simulink model "Shaddad_MCU"  (R2026b)
undefined symbols (not defined in the file): P, Ts
libraries: simulink x25
settings Model: Creator=aomar  LastModifiedBy=aomar

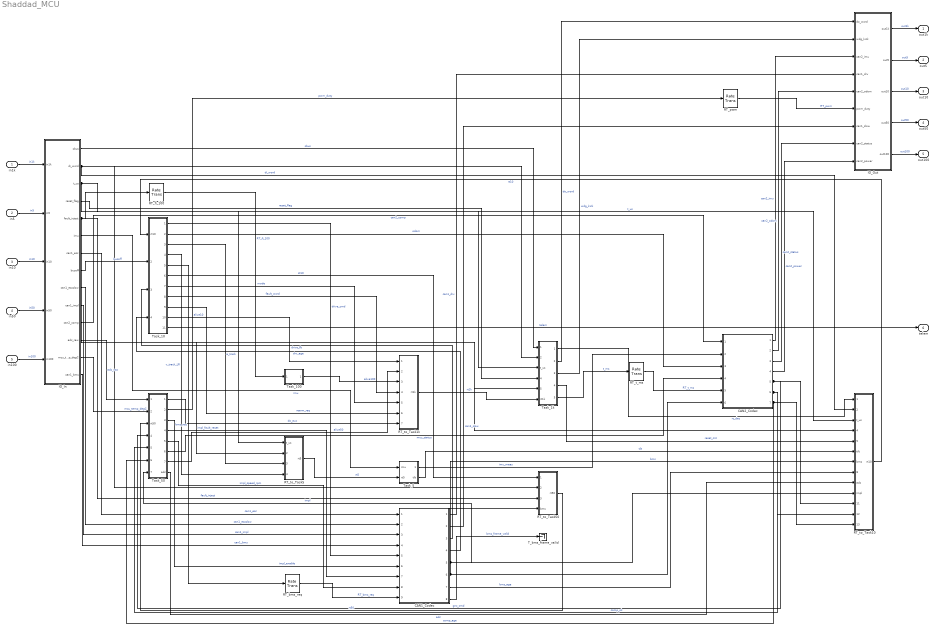
== system Shaddad_MCU ==
  in1k : Inport  OutDataTypeStr=Bus: Bus_McuIn1k  SampleTime=Ts.base  BusOutputAsStruct=on
  in5 : Inport  Port=2  OutDataTypeStr=Bus: Bus_McuIn5  SampleTime=Ts.imu  BusOutputAsStruct=on
  in10 : Inport  Port=3  OutDataTypeStr=Bus: Bus_McuIn10  SampleTime=Ts.ctrl  BusOutputAsStruct=on
  in50 : Inport  Port=4  OutDataTypeStr=Bus: Bus_McuIn50  SampleTime=Ts.comm  BusOutputAsStruct=on
  in100 : Inport  Port=5  OutDataTypeStr=Bus: Bus_McuIn100  SampleTime=Ts.hk  BusOutputAsStruct=on
  CAN1_Codec : Subsystem  ReferencedSubsystem=fw_can1_codec
  CAN2_Codec : Subsystem  ReferencedSubsystem=fw_can2_codec
  IO_In : Subsystem  Variant=on
  IO_Out : Subsystem  Variant=on
  RT_bms_req : RateTransition  OutPortSampleTime=Ts.comm
  RT_fi_100 : RateTransition  OutPortSampleTime=Ts.hk
  RT_pwm : RateTransition  OutPortSampleTime=Ts.ctrl
  RT_t_ms : RateTransition  OutPortSampleTime=Ts.comm
  RT_to_Task10 : Subsystem
  RT_to_Task1k : Subsystem
  RT_to_Task5 : Subsystem
  RT_to_Task50 : Subsystem
  T_bms_frame_valid : Terminator
  Task_10 : Subsystem  TreatAsAtomicUnit=on  SystemSampleTime=Ts.ctrl
  Task_100 : Subsystem  TreatAsAtomicUnit=on  SystemSampleTime=Ts.hk
  Task_1k : Subsystem  TreatAsAtomicUnit=on  SystemSampleTime=Ts.base
  Task_5 : Subsystem  TreatAsAtomicUnit=on  SystemSampleTime=Ts.imu
  Task_50 : Subsystem  TreatAsAtomicUnit=on  SystemSampleTime=Ts.comm
  out1k : Outport  OutDataTypeStr=Bus: Bus_McuOut1k  SampleTime=Ts.base  BusOutputAsStruct=on
  out5 : Outport  Port=2  OutDataTypeStr=Bus: Bus_McuOut5  SampleTime=Ts.imu  BusOutputAsStruct=on
  out10 : Outport  Port=3  OutDataTypeStr=Bus: Bus_McuOut10  SampleTime=Ts.ctrl  BusOutputAsStruct=on
  out50 : Outport  Port=4  OutDataTypeStr=Bus: Bus_McuOut50  SampleTime=Ts.comm  BusOutputAsStruct=on
  out100 : Outport  Port=5  OutDataTypeStr=Bus: Bus_McuOut100  SampleTime=Ts.hk  BusOutputAsStruct=on
  telem : Outport  Port=6  OutDataTypeStr=Bus: Bus_FwTelemetry  SampleTime=Ts.ctrl  BusOutputAsStruct=on
  wires:
  in1k/1 -> IO_In/1(in1k)  "in1k"
  in5/1 -> IO_In/2(in5)  "in5"
  in10/1 -> IO_In/3(in10)  "in10"
  in50/1 -> IO_In/4(in50)  "in50"
  in100/1 -> IO_In/5(in100)  "in100"
  IO_In/1(sbus) -> Task_1k/1(sbus)  "sbus"
  IO_In/2(di_word) -> RT_to_Task50/2(di_word), RT_to_Task10/2(di_word), Task_1k/2(di_word)  "di_word"
  IO_In/3(t_us) -> RT_to_Task5/1(t_us), RT_to_Task10/3(t_us), Task_1k/3(t_us)  "t_us"
  IO_In/4(reset_flag) -> Task_1k/4(reset_flag)  "reset_flag"
  IO_In/6(imu) -> Task_5/1(imu)  "imu"
  IO_In/7(can1_esc) -> CAN1_Codec/1  "can1_esc"
  IO_In/8(busoff) -> Task_10/2(busoff)  "busoff"
  IO_In/9(can1_escslow) -> CAN1_Codec/2  "can1_escslow"
  IO_In/10(can1_impl) -> CAN1_Codec/3  "can1_impl"
  IO_In/11(can2_comp) -> CAN2_Codec/1  "can2_comp"
  IO_In/13(mcu_temp_degC) -> Task_50/2(mcu_temp_degC)  "mcu_temp_degC"
  IO_In/14(can1_bms) -> CAN1_Codec/4  "can1_bms"
  RT_fi_100/1 -> Task_100/1(fault_inject)  "RT_fi_100"
  Task_10/1(drive_cmd) -> CAN1_Codec/5  "drive_cmd"
  Task_10/2(odom) -> CAN2_Codec/3  "odom"
  Task_10/3(a_track) -> RT_to_Task5/3(a_track)  "a_track"
  Task_10/4(v_track_LR) -> RT_to_Task5/4(v_track_LR)  "v_track_LR"
  Task_10/5(bms_req) -> RT_bms_req/1  "bms_req"
  Task_10/6(st10) -> RT_to_Task50/1(st10)  "st10"
  Task_10/7(mode) -> RT_to_Task1k/5(mode)  "mode"
  Task_10/8(fault_word) -> RT_to_Task1k/4(fault_word)  "fault_word"
  Task_10/9(rearm_req) -> RT_to_Task1k/6(rearm_req)  "rearm_req"
  Task_10/10(alive10) -> RT_to_Task1k/1(alive10)  "alive10"
  Task_10/11(telem) -> telem/1  "telem"
  Task_50/1(do_aux) -> RT_to_Task1k/7(do_aux)  "do_aux"
  Task_50/2(pwm_duty) -> RT_pwm/1  "pwm_duty"
  Task_50/3(impl_enable) -> CAN1_Codec/6  "impl_enable"
  Task_50/4(impl_fault_reset) -> CAN1_Codec/7  "impl_fault_reset"
  Task_50/5(impl_speed_rpm) -> CAN1_Codec/8  "impl_speed_rpm"
  Task_50/6(status) -> CAN2_Codec/4  "mcu_status"
  Task_50/7(alive50) -> RT_to_Task1k/2(alive50)  "alive50"
  Task_50/8(adc) -> RT_to_Task10/9(adc)  "adc"
  RT_bms_req/1 -> CAN1_Codec/9  "RT_bms_req"
  Task_100/1(alive100) -> RT_to_Task1k/3(alive100)  "alive100"
  RT_to_Task5/1(rt5) -> Task_5/2(rt5)  "rt5"
  RT_to_Task1k/1(rt1k) -> Task_1k/6(rt1k)  "rt1k"
  Task_5/1(imu_meas) -> CAN2_Codec/2  "imu_meas"
  Task_5/2(tilt) -> RT_to_Task10/6(tilt)  "tilt"
  CAN1_Codec/1 -> IO_Out/4(can1_drv)  "can1_drv"
  CAN1_Codec/2 -> IO_Out/7(can1_slow)  "can1_slow"
  CAN1_Codec/3 -> Task_10/3(drive_fb)  "drive_fb"
  CAN1_Codec/4 -> Task_10/4(drv_age)  "drv_age"
  CAN1_Codec/5 -> Task_50/7(impl), RT_to_Task10/10(impl)  "impl"
  CAN1_Codec/6 -> CAN2_Codec/6, RT_to_Task10/7(bms), RT_to_Task50/4(bms)  "bms"
  CAN1_Codec/7 -> RT_to_Task10/8(bms_age)  "bms_age"
  CAN1_Codec/8 -> T_bms_frame_valid/1  "bms_frame_valid"
  Task_1k/1(rc_dec) -> RT_to_Task10/1(rc_dec)  "rc_dec"
  Task_1k/2(do_word) -> IO_Out/1(do_word)  "do_word"
  Task_1k/3(wdg_kick) -> IO_Out/2(wdg_kick)  "wdg_kick"
  Task_1k/4(reset_cnt) -> RT_to_Task10/5(reset_cnt)  "reset_cnt"
  Task_1k/5(t_ms) -> RT_t_ms/1  "t_ms"
  RT_to_Task50/1(rt50) -> Task_50/3(rt50)  "rt50"
  RT_t_ms/1 -> CAN2_Codec/5  "RT_t_ms"
  RT_pwm/1 -> IO_Out/6(pwm_duty)  "RT_pwm"
  CAN2_Codec/1 -> IO_Out/3(can2_imu)  "can2_imu"
  CAN2_Codec/2 -> IO_Out/5(can2_odom)  "can2_odom"
  CAN2_Codec/3 -> IO_Out/8(can2_status)  "can2_status"
  CAN2_Codec/4 -> IO_Out/9(can2_power)  "can2_power"
  RT_to_Task10/1(rt10) -> Task_10/1(rt10)  "rt10"
  IO_Out/1(out1k) -> out1k/1  "out1k"
  IO_Out/2(out5) -> out5/1  "out5"
  IO_Out/3(out10) -> out10/1  "out10"
  IO_Out/4(out50) -> out50/1  "out50"
  IO_Out/5(out100) -> out100/1  "out100"
  CAN2_Codec/5 -> RT_to_Task10/11(gnc_cmd), Task_50/4(gnc_cmd)  "gnc_cmd"
  IO_In/5(fault_inject) -> RT_to_Task50/3(fault_inject), RT_to_Task5/2(fault_inject), RT_to_Task10/4(fault_inject), Task_1k/5(fault_inject), RT_fi_100/1  "fault_inject"
  IO_In/12(adc_raw) -> Task_50/1(adc_raw)  "adc_raw"
  CAN2_Codec/6 -> RT_to_Task10/12(comp_ok), Task_50/5(comp_ok)  "comp_ok"
  CAN2_Codec/7 -> RT_to_Task10/13(comp_age), Task_50/6(comp_age)  "comp_age"

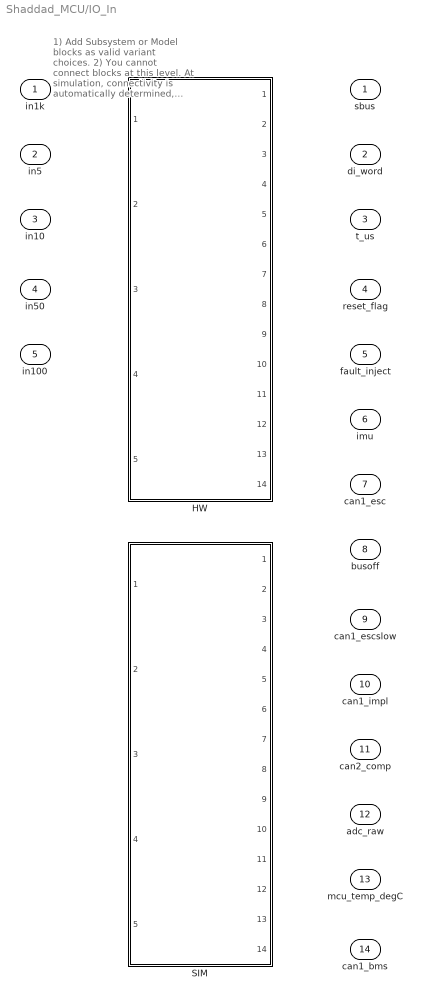
== system Shaddad_MCU/IO_In ==
  note: 1) Add Subsystem or Model blocks as valid variant choices.
      | 2) You cannot connect blocks at this level. At simulation, connectivity is automatically
      | determined, based on the active variant and port name matching.
  in1k : Inport
  in5 : Inport  Port=2
  in10 : Inport  Port=3
  in50 : Inport  Port=4
  in100 : Inport  Port=5
  HW : Subsystem  VariantControl=VC_TARGET == 1  ReferencedSubsystem=fw_io_in_hw
  SIM : Subsystem  VariantControl=VC_TARGET == 0  ReferencedSubsystem=fw_io_in_sim
  sbus : Outport
  di_word : Outport  Port=2
  t_us : Outport  Port=3
  reset_flag : Outport  Port=4
  fault_inject : Outport  Port=5
  imu : Outport  Port=6
  can1_esc : Outport  Port=7
  busoff : Outport  Port=8
  can1_escslow : Outport  Port=9
  can1_impl : Outport  Port=10
  can2_comp : Outport  Port=11
  adc_raw : Outport  Port=12
  mcu_temp_degC : Outport  Port=13
  can1_bms : Outport  Port=14

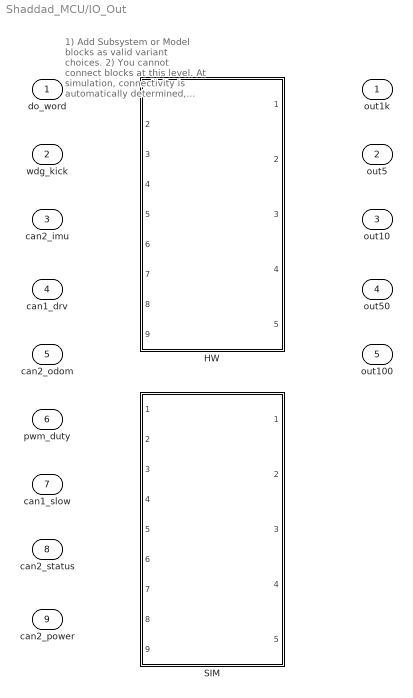
== system Shaddad_MCU/IO_Out ==
  note: 1) Add Subsystem or Model blocks as valid variant choices.
      | 2) You cannot connect blocks at this level. At simulation, connectivity is automatically
      | determined, based on the active variant and port name matching.
  do_word : Inport
  wdg_kick : Inport  Port=2
  can2_imu : Inport  Port=3
  can1_drv : Inport  Port=4
  can2_odom : Inport  Port=5
  pwm_duty : Inport  Port=6
  can1_slow : Inport  Port=7
  can2_status : Inport  Port=8
  can2_power : Inport  Port=9
  HW : Subsystem  VariantControl=VC_TARGET == 1  ReferencedSubsystem=fw_io_out_hw
  SIM : Subsystem  VariantControl=VC_TARGET == 0  ReferencedSubsystem=fw_io_out_sim
  out1k : Outport
  out5 : Outport  Port=2
  out10 : Outport  Port=3
  out50 : Outport  Port=4
  out100 : Outport  Port=5

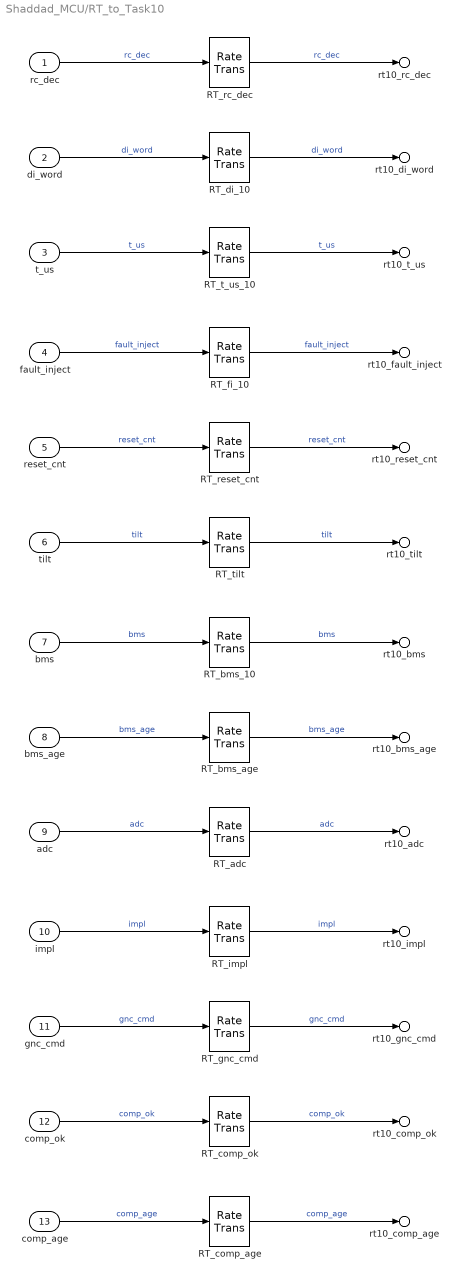
== system Shaddad_MCU/RT_to_Task10 ==
  rc_dec : Inport
  di_word : Inport  Port=2  OutDataTypeStr=uint16
  t_us : Inport  Port=3  OutDataTypeStr=uint32
  fault_inject : Inport  Port=4  OutDataTypeStr=uint32
  reset_cnt : Inport  Port=5  OutDataTypeStr=uint8
  tilt : Inport  Port=6
  bms : Inport  Port=7  OutDataTypeStr=Bus: Bus_BmsStatus
  bms_age : Inport  Port=8  OutDataTypeStr=single
  adc : Inport  Port=9
  impl : Inport  Port=10
  gnc_cmd : Inport  Port=11  OutDataTypeStr=Bus: Bus_GncCmd
  comp_ok : Inport  Port=12  OutDataTypeStr=boolean
  comp_age : Inport  Port=13  OutDataTypeStr=single
  RT_adc : RateTransition  OutPortSampleTime=Ts.ctrl
  RT_bms_10 : RateTransition  InitialCondition=P.ic.Bus_BmsStatus  OutPortSampleTime=Ts.ctrl
  RT_bms_age : RateTransition  OutPortSampleTime=Ts.ctrl
  RT_comp_age : RateTransition  OutPortSampleTime=Ts.ctrl
  RT_comp_ok : RateTransition  OutPortSampleTime=Ts.ctrl
  RT_di_10 : RateTransition  OutPortSampleTime=Ts.ctrl
  RT_fi_10 : RateTransition  OutPortSampleTime=Ts.ctrl
  RT_gnc_cmd : RateTransition  InitialCondition=P.ic.Bus_GncCmd  OutPortSampleTime=Ts.ctrl
  RT_impl : RateTransition  OutPortSampleTime=Ts.ctrl
  RT_rc_dec : RateTransition  OutPortSampleTime=Ts.ctrl
  RT_reset_cnt : RateTransition  OutPortSampleTime=Ts.ctrl
  RT_t_us_10 : RateTransition  OutPortSampleTime=Ts.ctrl
  RT_tilt : RateTransition  OutPortSampleTime=Ts.ctrl
  rt10_rc_dec : Outport  PortName=rt10  Element=rc_dec
  rt10_di_word : Outport  PortName=rt10  Element=di_word
  rt10_t_us : Outport  PortName=rt10  Element=t_us
  rt10_fault_inject : Outport  PortName=rt10  Element=fault_inject
  rt10_reset_cnt : Outport  PortName=rt10  Element=reset_cnt
  rt10_tilt : Outport  PortName=rt10  Element=tilt
  rt10_bms : Outport  PortName=rt10  Element=bms
  rt10_bms_age : Outport  PortName=rt10  Element=bms_age
  rt10_adc : Outport  PortName=rt10  Element=adc
  rt10_impl : Outport  PortName=rt10  Element=impl
  rt10_gnc_cmd : Outport  PortName=rt10  Element=gnc_cmd
  rt10_comp_ok : Outport  PortName=rt10  Element=comp_ok
  rt10_comp_age : Outport  PortName=rt10  Element=comp_age
  wires:
  rc_dec/1 -> RT_rc_dec/1  "rc_dec"
  di_word/1 -> RT_di_10/1  "di_word"
  t_us/1 -> RT_t_us_10/1  "t_us"
  fault_inject/1 -> RT_fi_10/1  "fault_inject"
  reset_cnt/1 -> RT_reset_cnt/1  "reset_cnt"
  tilt/1 -> RT_tilt/1  "tilt"
  bms/1 -> RT_bms_10/1  "bms"
  bms_age/1 -> RT_bms_age/1  "bms_age"
  adc/1 -> RT_adc/1  "adc"
  impl/1 -> RT_impl/1  "impl"
  gnc_cmd/1 -> RT_gnc_cmd/1  "gnc_cmd"
  comp_ok/1 -> RT_comp_ok/1  "comp_ok"
  comp_age/1 -> RT_comp_age/1  "comp_age"
  RT_rc_dec/1 -> rt10_rc_dec/1  "rc_dec"
  RT_di_10/1 -> rt10_di_word/1  "di_word"
  RT_t_us_10/1 -> rt10_t_us/1  "t_us"
  RT_fi_10/1 -> rt10_fault_inject/1  "fault_inject"
  RT_reset_cnt/1 -> rt10_reset_cnt/1  "reset_cnt"
  RT_tilt/1 -> rt10_tilt/1  "tilt"
  RT_bms_10/1 -> rt10_bms/1  "bms"
  RT_bms_age/1 -> rt10_bms_age/1  "bms_age"
  RT_adc/1 -> rt10_adc/1  "adc"
  RT_impl/1 -> rt10_impl/1  "impl"
  RT_gnc_cmd/1 -> rt10_gnc_cmd/1  "gnc_cmd"
  RT_comp_ok/1 -> rt10_comp_ok/1  "comp_ok"
  RT_comp_age/1 -> rt10_comp_age/1  "comp_age"

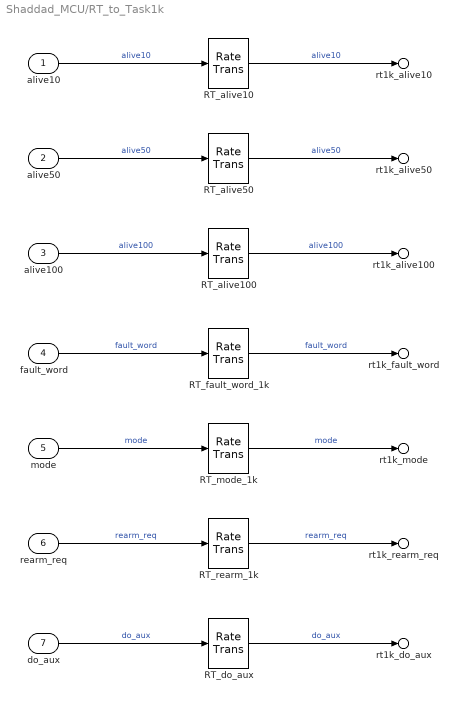
== system Shaddad_MCU/RT_to_Task1k ==
  alive10 : Inport  OutDataTypeStr=uint8
  alive50 : Inport  Port=2  OutDataTypeStr=uint8
  alive100 : Inport  Port=3  OutDataTypeStr=uint8
  fault_word : Inport  Port=4  OutDataTypeStr=uint32
  mode : Inport  Port=5  OutDataTypeStr=uint8
  rearm_req : Inport  Port=6  OutDataTypeStr=boolean
  do_aux : Inport  Port=7  OutDataTypeStr=uint32
  RT_alive10 : RateTransition  OutPortSampleTime=Ts.base
  RT_alive100 : RateTransition  OutPortSampleTime=Ts.base
  RT_alive50 : RateTransition  OutPortSampleTime=Ts.base
  RT_do_aux : RateTransition  OutPortSampleTime=Ts.base
  RT_fault_word_1k : RateTransition  OutPortSampleTime=Ts.base
  RT_mode_1k : RateTransition  OutPortSampleTime=Ts.base
  RT_rearm_1k : RateTransition  OutPortSampleTime=Ts.base
  rt1k_alive10 : Outport  PortName=rt1k  Element=alive10
  rt1k_alive50 : Outport  PortName=rt1k  Element=alive50
  rt1k_alive100 : Outport  PortName=rt1k  Element=alive100
  rt1k_fault_word : Outport  PortName=rt1k  Element=fault_word
  rt1k_mode : Outport  PortName=rt1k  Element=mode
  rt1k_rearm_req : Outport  PortName=rt1k  Element=rearm_req
  rt1k_do_aux : Outport  PortName=rt1k  Element=do_aux
  wires:
  alive10/1 -> RT_alive10/1  "alive10"
  alive50/1 -> RT_alive50/1  "alive50"
  alive100/1 -> RT_alive100/1  "alive100"
  fault_word/1 -> RT_fault_word_1k/1  "fault_word"
  mode/1 -> RT_mode_1k/1  "mode"
  rearm_req/1 -> RT_rearm_1k/1  "rearm_req"
  do_aux/1 -> RT_do_aux/1  "do_aux"
  RT_alive10/1 -> rt1k_alive10/1  "alive10"
  RT_alive50/1 -> rt1k_alive50/1  "alive50"
  RT_alive100/1 -> rt1k_alive100/1  "alive100"
  RT_fault_word_1k/1 -> rt1k_fault_word/1  "fault_word"
  RT_mode_1k/1 -> rt1k_mode/1  "mode"
  RT_rearm_1k/1 -> rt1k_rearm_req/1  "rearm_req"
  RT_do_aux/1 -> rt1k_do_aux/1  "do_aux"

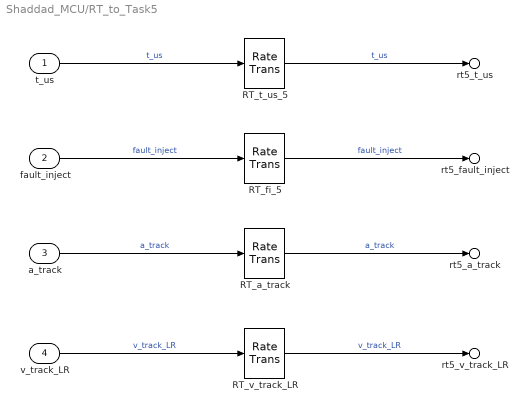
== system Shaddad_MCU/RT_to_Task5 ==
  t_us : Inport  OutDataTypeStr=uint32
  fault_inject : Inport  Port=2  OutDataTypeStr=uint32
  a_track : Inport  Port=3  OutDataTypeStr=single
  v_track_LR : Inport  Port=4  OutDataTypeStr=single
  RT_a_track : RateTransition  OutPortSampleTime=Ts.imu
  RT_fi_5 : RateTransition  OutPortSampleTime=Ts.imu
  RT_t_us_5 : RateTransition  OutPortSampleTime=Ts.imu
  RT_v_track_LR : RateTransition  OutPortSampleTime=Ts.imu
  rt5_t_us : Outport  PortName=rt5  Element=t_us
  rt5_fault_inject : Outport  PortName=rt5  Element=fault_inject
  rt5_a_track : Outport  PortName=rt5  Element=a_track
  rt5_v_track_LR : Outport  PortName=rt5  Element=v_track_LR
  wires:
  t_us/1 -> RT_t_us_5/1  "t_us"
  fault_inject/1 -> RT_fi_5/1  "fault_inject"
  a_track/1 -> RT_a_track/1  "a_track"
  v_track_LR/1 -> RT_v_track_LR/1  "v_track_LR"
  RT_t_us_5/1 -> rt5_t_us/1  "t_us"
  RT_fi_5/1 -> rt5_fault_inject/1  "fault_inject"
  RT_a_track/1 -> rt5_a_track/1  "a_track"
  RT_v_track_LR/1 -> rt5_v_track_LR/1  "v_track_LR"

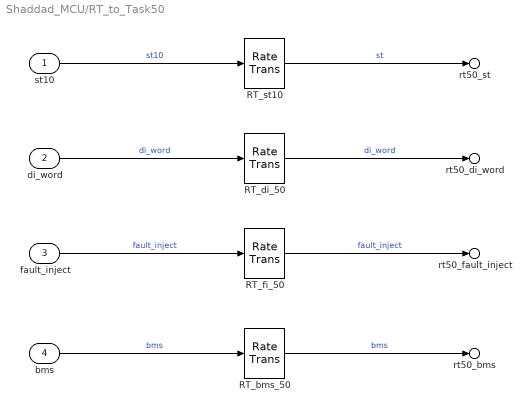
== system Shaddad_MCU/RT_to_Task50 ==
  st10 : Inport
  di_word : Inport  Port=2  OutDataTypeStr=uint16
  fault_inject : Inport  Port=3  OutDataTypeStr=uint32
  bms : Inport  Port=4  OutDataTypeStr=Bus: Bus_BmsStatus
  RT_bms_50 : RateTransition  InitialCondition=P.ic.Bus_BmsStatus  OutPortSampleTime=Ts.comm
  RT_di_50 : RateTransition  OutPortSampleTime=Ts.comm
  RT_fi_50 : RateTransition  OutPortSampleTime=Ts.comm
  RT_st10 : RateTransition  OutPortSampleTime=Ts.comm
  rt50_st : Outport  PortName=rt50  Element=st
  rt50_di_word : Outport  PortName=rt50  Element=di_word
  rt50_fault_inject : Outport  PortName=rt50  Element=fault_inject
  rt50_bms : Outport  PortName=rt50  Element=bms
  wires:
  st10/1 -> RT_st10/1  "st10"
  di_word/1 -> RT_di_50/1  "di_word"
  fault_inject/1 -> RT_fi_50/1  "fault_inject"
  bms/1 -> RT_bms_50/1  "bms"
  RT_st10/1 -> rt50_st/1  "st"
  RT_di_50/1 -> rt50_di_word/1  "di_word"
  RT_fi_50/1 -> rt50_fault_inject/1  "fault_inject"
  RT_bms_50/1 -> rt50_bms/1  "bms"

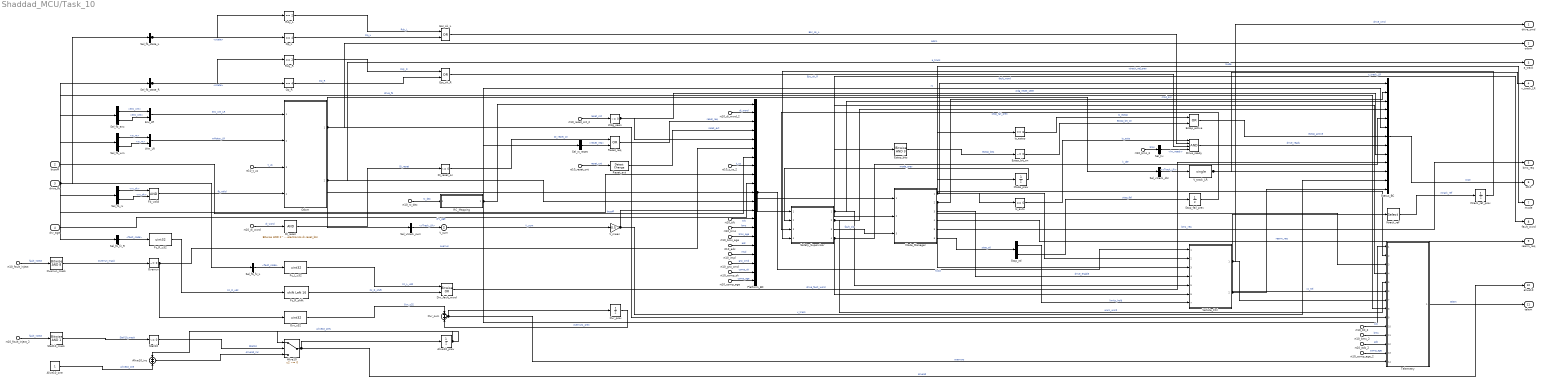
== system Shaddad_MCU/Task_10 ==
  rt10_rc_dec : Inport  PortName=rt10  Element=rc_dec
  rt10_t_us : Inport  PortName=rt10  Element=t_us
  rt10_t_us_2 : Inport  PortName=rt10  Element=t_us
  rt10_di_word : Inport  PortName=rt10  Element=di_word
  rt10_di_word_2 : Inport  PortName=rt10  Element=di_word
  rt10_reset_cnt : Inport  PortName=rt10  Element=reset_cnt
  rt10_reset_cnt_2 : Inport  PortName=rt10  Element=reset_cnt
  rt10_fault_inject : Inport  PortName=rt10  Element=fault_inject
  rt10_fault_inject_2 : Inport  PortName=rt10  Element=fault_inject
  rt10_tilt : Inport  PortName=rt10  Element=tilt
  rt10_tilt_2 : Inport  PortName=rt10  Element=tilt
  rt10_bms : Inport  PortName=rt10  Element=bms
  rt10_bms_2 : Inport  PortName=rt10  Element=bms
  rt10_bms_3 : Inport  PortName=rt10  Element=bms
  rt10_bms_age : Inport  PortName=rt10  Element=bms_age
  rt10_adc : Inport  PortName=rt10  Element=adc
  rt10_adc_2 : Inport  PortName=rt10  Element=adc
  rt10_impl : Inport  PortName=rt10  Element=impl
  rt10_gnc_cmd : Inport  PortName=rt10  Element=gnc_cmd
  rt10_comp_ok : Inport  PortName=rt10  Element=comp_ok
  rt10_comp_age : Inport  PortName=rt10  Element=comp_age
  rt10_comp_age_2 : Inport  PortName=rt10  Element=comp_age
  busoff : Inport  Port=2  OutDataTypeStr=boolean
  drive_fb : Inport  Port=3  OutDataTypeStr=Bus: Bus_DriveFb
  drv_age : Inport  Port=4  OutDataTypeStr=single
  Alive10 : Switch  Criteria=u2 ~= 0  SaturateOnIntegerOverflow=off  InputSameDT=off
  Alive10_inc : Sum  OutDataTypeStr=uint8
  Alive10_one : Constant  OutDataTypeStr=uint8  SampleTime=-1
  Alive10_prev : UnitDelay  SampleTime=-1
  DI_reset : simulink/Logic and Bit Operations/Bitwise Operator  logicop=AND  UseBitMask=on  BitMask=2^P.electronics.di.reset_btn  BitMaskRealWorld=Stored Integer
  DI_reset_on : simulink/Logic and Bit Operations/Compare To Zero  relop=~=  OutDataTypeStr=boolean
  Drive_ready : Logic  Inputs=4  AllPortsSameDT=off  OutDataTypeStr=boolean
  Drv_fault_word : simulink/Logic and Bit Operations/Bitwise Operator  logicop=OR  UseBitMask=off  NumInputPorts=2  BitMask=bin2dec('11011001')  BitMaskRealWorld=Stored Integer
  Enc_LR : Concatenate
  Esc_ok_L : Logic  Operator=OR  AllPortsSameDT=off  OutDataTypeStr=boolean
  Esc_ok_R : Logic  Operator=OR  AllPortsSameDT=off  OutDataTypeStr=boolean
  Estop_active : Logic  Operator=OR  AllPortsSameDT=off  OutDataTypeStr=boolean
  Estop_bit_on : simulink/Logic and Bit Operations/Compare To Zero  relop=~=  OutDataTypeStr=boolean
  Estop_bits : simulink/Logic and Bit Operations/Bitwise Operator  logicop=AND  UseBitMask=on  BitMask=3  BitMaskRealWorld=Stored Integer
  Fb_valid : Logic  AllPortsSameDT=off  OutDataTypeStr=boolean
  Fc_L_u32 : DataTypeConversion  OutDataTypeStr=uint32  RndMeth=Round
  Fc_R_shift : ArithShift  BitShiftNumber=16  BitShiftDirection=Left
  Fc_R_u32 : DataTypeConversion  OutDataTypeStr=uint32  RndMeth=Round
  Is_auto : simulink/Logic and Bit Operations/Compare To Constant  relop===  const=6  OutDataTypeStr=boolean
  Is_estop : simulink/Logic and Bit Operations/Compare To Constant  relop===  const=8  OutDataTypeStr=boolean
  Mode_Manager : Subsystem  ReferencedSubsystem=fw_mode_manager
  Mode_prev : UnitDelay  SampleTime=-1
  Odom : Subsystem  ReferencedSubsystem=sens_odom_compute
  Op_L : simulink/Logic and Bit Operations/Compare To Constant  relop===  const=4  OutDataTypeStr=boolean
  Op_R : simulink/Logic and Bit Operations/Compare To Constant  relop===  const=4  OutDataTypeStr=boolean
  Overrun : simulink/Logic and Bit Operations/Compare To Zero  relop=~=  OutDataTypeStr=boolean
  Overrun_mask : simulink/Logic and Bit Operations/Bitwise Operator  logicop=AND  UseBitMask=on  BitMask=8  BitMaskRealWorld=Stored Integer
  Ovr_prev : UnitDelay  SampleTime=-1
  Ovr_sum : Sum  OutDataTypeStr=uint32  SaturateOnIntegerOverflow=on
  Ovr_u32 : DataTypeConversion  OutDataTypeStr=uint32  RndMeth=Round
  Platform_BC : BusCreator  Inputs=21
  RC_Mapping : Subsystem  ReferencedSubsystem=fw_rc_mapping
  Rdy_L : simulink/Logic and Bit Operations/Compare To Constant  relop===  const=2  OutDataTypeStr=boolean
  Rdy_R : simulink/Logic and Bit Operations/Compare To Constant  relop===  const=2  OutDataTypeStr=boolean
  Reset_evt : simulink/Logic and Bit Operations/Detect Change  vinit=0  OutDataTypeStr=boolean
  Reset_req : Logic  Operator=OR  AllPortsSameDT=off  OutDataTypeStr=boolean
  Safety_Supervisor : Subsystem  ReferencedSubsystem=fw_safety_supervisor
  Sel_fb_enc : BusSelector  OutputSignals=L.enc_cnt,R.enc_cnt
  Sel_fb_fc_L : BusSelector  OutputSignals=L.fault_code
  Sel_fb_fc_R : BusSelector  OutputSignals=R.fault_code
  Sel_fb_rx : BusSelector  OutputSignals=L.rx_ok,R.rx_ok
  Sel_fb_state_L : BusSelector  OutputSignals=L.state
  Sel_fb_state_R : BusSelector  OutputSignals=R.state
  Sel_fb_wm : BusSelector  OutputSignals=L.w_m,R.w_m
  Sel_hv : BusSelector  OutputSignals=hv_ready
  Sel_rc_reset : BusSelector  OutputSignals=reset_req
  Sel_vtrack_dtc : BusSelector  OutputSignals=vTrack_LR
  Sel_vtrack_sum : BusSelector  OutputSignals=vTrack_LR
  Stall10 : simulink/Logic and Bit Operations/Compare To Zero  relop=~=  OutDataTypeStr=boolean
  Stall10_mask : simulink/Logic and Bit Operations/Bitwise Operator  logicop=AND  UseBitMask=on  BitMask=1  BitMaskRealWorld=Stored Integer
  Status_BC : BusCreator  Inputs=13
  Stop_ctl : Demux  Outputs=2
  Stop_fail_prev : UnitDelay  InitialCondition=false  SampleTime=-1
  Telemetry : Subsystem  ReferencedSubsystem=fw_telemetry
  V_mean : Gain  Gain=0.5
  V_sum : Sum  Inputs=+
  V_track_LR : DataTypeConversion  OutDataTypeStr=single  RndMeth=Round
  Vehicle_Ctrl : Subsystem  ReferencedSubsystem=fw_vehicle_ctrl
  Vtrack_ref : Selector  InputPortWidth=11  IndexOptions=Index vector (dialog)  Indices=[8 9]  OutputSizes=1
  Vtrack_ref_prev : UnitDelay  InitialCondition=[0 0]  SampleTime=-1
  Wdg_seen : simulink/Logic and Bit Operations/Compare To Zero  relop=~=  OutDataTypeStr=boolean
  Wm_LR : Concatenate
  drive_cmd : Outport
  odom : Outport  Port=2
  a_track : Outport  Port=3
  v_track_LR : Outport  Port=4
  bms_req : Outport  Port=5
  st10 : Outport  Port=6
  mode : Outport  Port=7
  fault_word : Outport  Port=8
  rearm_req : Outport  Port=9
  alive10 : Outport  Port=10
  telem : Outport  Port=11
  wires:
  rt10_fault_inject/1 -> Overrun_mask/1  "fault_inject"
  rt10_fault_inject_2/1 -> Stall10_mask/1  "fault_inject"
  busoff/1 -> Platform_BC/7  "busoff"
  drive_fb/1 -> Sel_fb_state_L/1, Telemetry/8, Sel_fb_state_R/1, Sel_fb_fc_L/1, Sel_fb_enc/1, Sel_fb_fc_R/1, Sel_fb_wm/1, Sel_fb_rx/1, Platform_BC/9  "drive_fb"
  drv_age/1 -> Platform_BC/10  "drv_age"
  Alive10_one/1 -> Alive10_inc/2  "Alive10_one"
  Overrun_mask/1 -> Overrun/1  "Overrun_mask"
  Stall10_mask/1 -> Stall10/1  "Stall10_mask"
  Sel_fb_enc/1 -> Enc_LR/1  "<enc_cnt>"
  Sel_fb_enc/2 -> Enc_LR/2  "<enc_cnt>"
  Sel_fb_wm/1 -> Wm_LR/1  "<w_m>"
  Sel_fb_wm/2 -> Wm_LR/2  "<w_m>"
  Sel_fb_rx/1 -> Fb_valid/1  "<rx_ok>"
  Sel_fb_rx/2 -> Fb_valid/2  "<rx_ok>"
  Sel_fb_fc_R/1 -> Fc_R_u32/1  "<fault_code>"
  Sel_fb_state_L/1 -> Rdy_L/1, Op_L/1  "<state>"
  Sel_fb_state_R/1 -> Rdy_R/1, Op_R/1  "<state>"
  Enc_LR/1 -> Odom/1  "enc_cnt_LR"
  Wm_LR/1 -> Odom/2  "wMotor_LR"
  Alive10_inc/1 -> Alive10/3  "Alive10_inc"
  Fb_valid/1 -> Odom/4  "fb_valid"
  Overrun/1 -> Platform_BC/6, Ovr_u32/1  "overrun"
  Stall10/1 -> Alive10/2  "Stall10"
  Fc_R_u32/1 -> Fc_R_shift/1  "Fc_R_u32"
  rt10_t_us/1 -> Odom/3  "t_us"
  rt10_di_word/1 -> DI_reset/1  "di_word"
  Sel_fb_fc_L/1 -> Fc_L_u32/1  "<fault_code>"
  Rdy_L/1 -> Esc_ok_L/1  "Rdy_L"
  Op_L/1 -> Esc_ok_L/2  "Op_L"
  Rdy_R/1 -> Esc_ok_R/1  "Rdy_R"
  Op_R/1 -> Esc_ok_R/2  "Op_R"
  DI_reset/1 -> DI_reset_on/1  "DI_reset"
  Alive10/1 -> alive10/1, Alive10_prev/1  "alive10"
  Fc_L_u32/1 -> Drv_fault_word/1  "Fc_L_u32"
  Ovr_u32/1 -> Ovr_sum/1  "Ovr_u32"
  Fc_R_shift/1 -> Drv_fault_word/2  "Fc_R_shift"
  Odom/1 -> Telemetry/9, Sel_vtrack_sum/1, odom/1, Platform_BC/11, Sel_vtrack_dtc/1  "odom"
  Odom/2 -> a_track/1, Platform_BC/12  "a_track"
  rt10_rc_dec/1 -> RC_Mapping/1  "rc_dec"
  Sel_vtrack_sum/1 -> V_sum/1  "<vTrack_LR>"
  V_sum/1 -> V_mean/1  "V_sum"
  Ovr_sum/1 -> Telemetry/14, Ovr_prev/1  "overruns"
  Esc_ok_L/1 -> Drive_ready/2  "Esc_ok_L"
  Esc_ok_R/1 -> Drive_ready/3  "Esc_ok_R"
  DI_reset_on/1 -> Reset_req/1  "DI_reset_on"
  Alive10_prev/1 -> Alive10_inc/1, Alive10/1  "Alive10_prev"
  Drv_fault_word/1 -> Status_BC/10  "drive_fault_word"
  RC_Mapping/1 -> Platform_BC/1, Status_BC/6, Sel_rc_reset/1, Telemetry/1  "rc"
  rt10_reset_cnt_2/1 -> Wdg_seen/1  "reset_cnt"
  Sel_rc_reset/1 -> Reset_req/2  "<reset_req>"
  rt10_reset_cnt/1 -> Reset_evt/1  "reset_cnt"
  Wdg_seen/1 -> Status_BC/9, Platform_BC/5  "wdg_reset_seen"
  Reset_req/1 -> Platform_BC/3  "reset_req"
  V_mean/1 -> Status_BC/12, Platform_BC/13  "v_track"
  Ovr_prev/1 -> Ovr_sum/2  "overruns_prev"
  Reset_evt/1 -> Platform_BC/4  "reset_evt"
  rt10_di_word_2/1 -> Platform_BC/2  "di_word"
  rt10_t_us_2/1 -> Platform_BC/8  "t_us"
  rt10_tilt/1 -> Platform_BC/14  "tilt"
  rt10_bms/1 -> Platform_BC/15  "bms"
  rt10_bms_age/1 -> Platform_BC/16  "bms_age"
  rt10_adc/1 -> Platform_BC/17  "adc"
  rt10_impl/1 -> Platform_BC/18  "impl"
  rt10_gnc_cmd/1 -> Platform_BC/19  "gnc_cmd"
  rt10_comp_ok/1 -> Platform_BC/20  "comp_ok"
  rt10_comp_age/1 -> Platform_BC/21  "comp_age"
  Platform_BC/1 -> Vehicle_Ctrl/1, Safety_Supervisor/1, Mode_Manager/1  "fw10"
  Safety_Supervisor/3 -> Mode_Manager/3  "fault_cls"
  Estop_bits/1 -> Estop_bit_on/1  "Estop_bits"
  Mode_Manager/3 -> Vehicle_Ctrl/4  "drive_enable"
  Mode_Manager/4 -> rearm_req/1  "rearm_req"
  Mode_Manager/5 -> bms_req/1  "bms_req"
  Mode_Manager/6 -> Stop_ctl/1  "stop_ctl"
  Stop_ctl/1 -> Vehicle_Ctrl/7  "limits_hold"
  Stop_ctl/2 -> Stop_fail_prev/1  "stop_fail"
  Is_estop/1 -> Estop_active/1  "Is_estop"
  Estop_bit_on/1 -> Estop_active/2  "Estop_bit_on"
  Is_auto/1 -> Drive_ready/1  "Is_auto"
  Mode_prev/1 -> Safety_Supervisor/2  "mode_prev"
  rt10_bms_3/1 -> Sel_hv/1  "bms"
  Sel_hv/1 -> Drive_ready/4  "<hv_ready>"
  Sel_vtrack_dtc/1 -> V_track_LR/1  "<vTrack_LR>"
  Estop_active/1 -> Status_BC/7  "estop_active"
  Drive_ready/1 -> Status_BC/8  "drive_ready"
  Stop_fail_prev/1 -> Safety_Supervisor/3  "stop_fail_prev"
  V_track_LR/1 -> v_track_LR/1, Status_BC/11  "v_track_LR"
  rt10_tilt_2/1 -> Telemetry/10  "tilt"
  rt10_bms_2/1 -> Telemetry/11  "bms"
  rt10_adc_2/1 -> Telemetry/12  "adc"
  rt10_comp_age_2/1 -> Telemetry/13  "comp_age"
  Status_BC/1 -> st10/1  "st10"
  Vtrack_ref/1 -> Vtrack_ref_prev/1  "vtrack_ref"
  Telemetry/1 -> telem/1  "telem"
  Vtrack_ref_prev/1 -> Safety_Supervisor/4  "vtrack_ref_prev"
  Vehicle_Ctrl/1 -> Telemetry/7, drive_cmd/1  "drive_cmd"
  Vehicle_Ctrl/2 -> Status_BC/13, Vtrack_ref/1, Telemetry/6  "vc_tel"
  Mode_Manager/1 -> Status_BC/1, Vehicle_Ctrl/2, Is_estop/1, Telemetry/2, Mode_prev/1, Is_auto/1, mode/1  "mode"
  Mode_Manager/2 -> Status_BC/2, Vehicle_Ctrl/3, Telemetry/3  "cmd_src"
  Safety_Supervisor/1 -> Status_BC/3, Vehicle_Ctrl/5, Estop_bits/1, Telemetry/4, fault_word/1, Mode_Manager/2  "fault_word"
  Safety_Supervisor/2 -> Status_BC/4, Telemetry/5  "warn_word"
  Safety_Supervisor/4 -> Status_BC/5, Vehicle_Ctrl/6  "k_der"

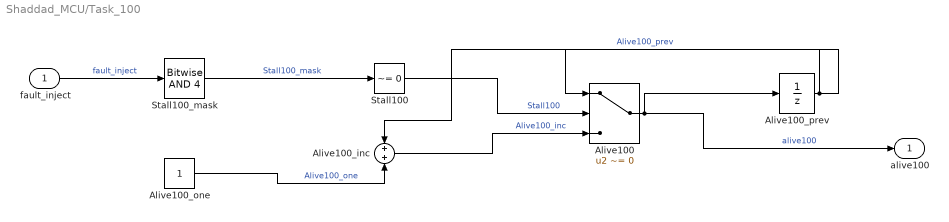
== system Shaddad_MCU/Task_100 ==
  fault_inject : Inport  OutDataTypeStr=uint32
  Alive100 : Switch  Criteria=u2 ~= 0  SaturateOnIntegerOverflow=off  InputSameDT=off
  Alive100_inc : Sum  OutDataTypeStr=uint8
  Alive100_one : Constant  OutDataTypeStr=uint8  SampleTime=-1
  Alive100_prev : UnitDelay  SampleTime=-1
  Stall100 : simulink/Logic and Bit Operations/Compare To Zero  relop=~=  OutDataTypeStr=boolean
  Stall100_mask : simulink/Logic and Bit Operations/Bitwise Operator  logicop=AND  UseBitMask=on  BitMask=4  BitMaskRealWorld=Stored Integer
  alive100 : Outport
  wires:
  fault_inject/1 -> Stall100_mask/1  "fault_inject"
  Alive100_one/1 -> Alive100_inc/2  "Alive100_one"
  Stall100_mask/1 -> Stall100/1  "Stall100_mask"
  Alive100_inc/1 -> Alive100/3  "Alive100_inc"
  Stall100/1 -> Alive100/2  "Stall100"
  Alive100/1 -> alive100/1, Alive100_prev/1  "alive100"
  Alive100_prev/1 -> Alive100_inc/1, Alive100/1  "Alive100_prev"

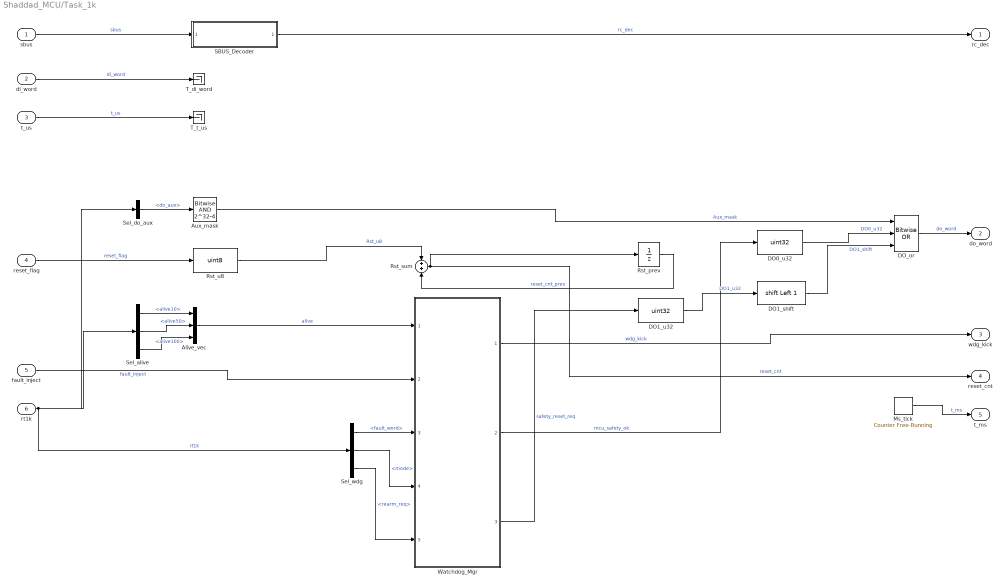
== system Shaddad_MCU/Task_1k ==
  sbus : Inport  OutDataTypeStr=Bus: Bus_SbusStream
  di_word : Inport  Port=2  OutDataTypeStr=uint16
  t_us : Inport  Port=3  OutDataTypeStr=uint32
  reset_flag : Inport  Port=4  OutDataTypeStr=boolean
  fault_inject : Inport  Port=5  OutDataTypeStr=uint32
  rt1k : Inport  Port=6
  Alive_vec : Concatenate  NumInputs=3
  Aux_mask : simulink/Logic and Bit Operations/Bitwise Operator  logicop=AND  UseBitMask=on  BitMask=2^32-4  BitMaskRealWorld=Stored Integer
  DO0_u32 : DataTypeConversion  OutDataTypeStr=uint32  RndMeth=Round
  DO1_shift : ArithShift  BitShiftNumber=1  BitShiftDirection=Left
  DO1_u32 : DataTypeConversion  OutDataTypeStr=uint32  RndMeth=Round
  DO_or : simulink/Logic and Bit Operations/Bitwise Operator  logicop=OR  UseBitMask=off  NumInputPorts=3  BitMask=bin2dec('11011001')  BitMaskRealWorld=Stored Integer
  Ms_tick : simulink/Sources/Counter Free-Running  NumBits=32  tsamp=Ts.base
  Rst_prev : UnitDelay  SampleTime=-1
  Rst_sum : Sum  OutDataTypeStr=uint8
  Rst_u8 : DataTypeConversion  OutDataTypeStr=uint8  RndMeth=Round
  SBUS_Decoder : Subsystem  ReferencedSubsystem=fw_sbus_decoder
  Sel_alive : BusSelector  OutputSignals=alive10,alive50,alive100
  Sel_do_aux : BusSelector  OutputSignals=do_aux
  Sel_wdg : BusSelector  OutputSignals=fault_word,mode,rearm_req
  T_di_word : Terminator
  T_t_us : Terminator
  Watchdog_Mgr : Subsystem  ReferencedSubsystem=fw_watchdog_mgr
  rc_dec : Outport
  do_word : Outport  Port=2
  wdg_kick : Outport  Port=3
  reset_cnt : Outport  Port=4
  t_ms : Outport  Port=5
  wires:
  sbus/1 -> SBUS_Decoder/1  "sbus"
  di_word/1 -> T_di_word/1  "di_word"
  t_us/1 -> T_t_us/1  "t_us"
  reset_flag/1 -> Rst_u8/1  "reset_flag"
  fault_inject/1 -> Watchdog_Mgr/2  "fault_inject"
  rt1k/1 -> Sel_do_aux/1, Sel_alive/1, Sel_wdg/1  "rt1k"
  Sel_do_aux/1 -> Aux_mask/1  "<do_aux>"
  Sel_alive/1 -> Alive_vec/1  "<alive10>"
  Sel_alive/2 -> Alive_vec/2  "<alive50>"
  Sel_alive/3 -> Alive_vec/3  "<alive100>"
  Alive_vec/1 -> Watchdog_Mgr/1  "alive"
  Aux_mask/1 -> DO_or/1  "Aux_mask"
  Rst_u8/1 -> Rst_sum/1  "Rst_u8"
  SBUS_Decoder/1 -> rc_dec/1  "rc_dec"
  Sel_wdg/1 -> Watchdog_Mgr/3  "<fault_word>"
  Sel_wdg/2 -> Watchdog_Mgr/4  "<mode>"
  Sel_wdg/3 -> Watchdog_Mgr/5  "<rearm_req>"
  Rst_sum/1 -> reset_cnt/1, Rst_prev/1  "reset_cnt"
  Watchdog_Mgr/1 -> wdg_kick/1  "wdg_kick"
  Watchdog_Mgr/2 -> DO0_u32/1  "mcu_safety_ok"
  Watchdog_Mgr/3 -> DO1_u32/1  "safety_reset_req"
  Rst_prev/1 -> Rst_sum/2  "reset_cnt_prev"
  DO1_u32/1 -> DO1_shift/1  "DO1_u32"
  DO0_u32/1 -> DO_or/2  "DO0_u32"
  DO1_shift/1 -> DO_or/3  "DO1_shift"
  Ms_tick/1 -> t_ms/1  "t_ms"
  DO_or/1 -> do_word/1  "do_word"

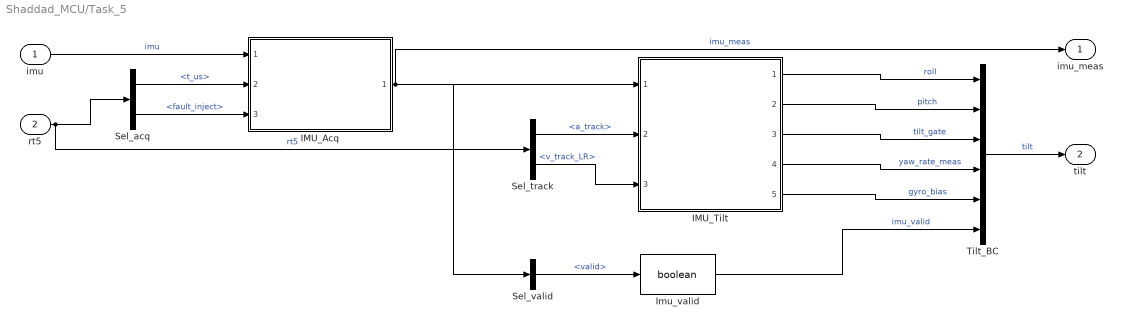
== system Shaddad_MCU/Task_5 ==
  imu : Inport  OutDataTypeStr=Bus: Bus_ImuRaw
  rt5 : Inport  Port=2
  IMU_Acq : Subsystem  ReferencedSubsystem=sens_acq_imu
  IMU_Tilt : Subsystem  ReferencedSubsystem=fw_imu_tilt
  Imu_valid : DataTypeConversion  OutDataTypeStr=boolean  RndMeth=Round
  Sel_acq : BusSelector  OutputSignals=t_us,fault_inject
  Sel_track : BusSelector  OutputSignals=a_track,v_track_LR
  Sel_valid : BusSelector  OutputSignals=valid
  Tilt_BC : BusCreator  Inputs=6
  imu_meas : Outport
  tilt : Outport  Port=2
  wires:
  imu/1 -> IMU_Acq/1  "imu"
  rt5/1 -> Sel_acq/1, Sel_track/1  "rt5"
  Sel_acq/1 -> IMU_Acq/2  "<t_us>"
  Sel_acq/2 -> IMU_Acq/3  "<fault_inject>"
  IMU_Acq/1 -> Sel_valid/1, imu_meas/1, IMU_Tilt/1  "imu_meas"
  Sel_track/1 -> IMU_Tilt/2  "<a_track>"
  Sel_track/2 -> IMU_Tilt/3  "<v_track_LR>"
  Sel_valid/1 -> Imu_valid/1  "<valid>"
  Imu_valid/1 -> Tilt_BC/6  "imu_valid"
  IMU_Tilt/1 -> Tilt_BC/1  "roll"
  IMU_Tilt/2 -> Tilt_BC/2  "pitch"
  IMU_Tilt/3 -> Tilt_BC/3  "tilt_gate"
  IMU_Tilt/4 -> Tilt_BC/4  "yaw_rate_meas"
  IMU_Tilt/5 -> Tilt_BC/5  "gyro_bias"
  Tilt_BC/1 -> tilt/1  "tilt"

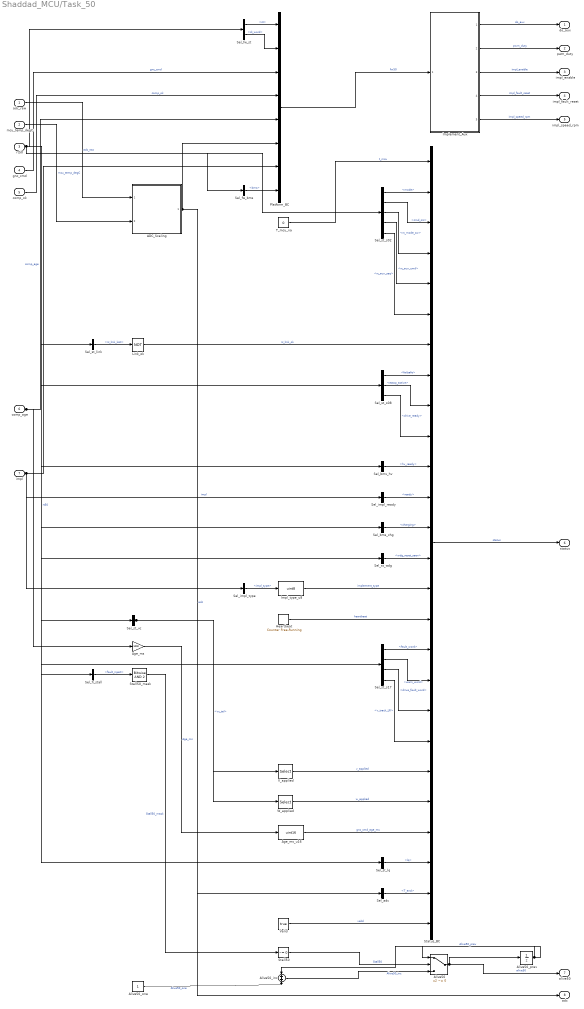
== system Shaddad_MCU/Task_50 ==
  adc_raw : Inport  OutDataTypeStr=uint16
  mcu_temp_degC : Inport  Port=2  OutDataTypeStr=single
  rt50 : Inport  Port=3
  gnc_cmd : Inport  Port=4  OutDataTypeStr=Bus: Bus_GncCmd
  comp_ok : Inport  Port=5  OutDataTypeStr=boolean
  comp_age : Inport  Port=6  OutDataTypeStr=single
  impl : Inport  Port=7
  ADC_Scaling : Subsystem  ReferencedSubsystem=fw_adc_scaling
  Age_ms : Gain  Gain=1000
  Age_ms_u16 : DataTypeConversion  OutDataTypeStr=uint16  RndMeth=Round
  Alive50 : Switch  Criteria=u2 ~= 0  SaturateOnIntegerOverflow=off  InputSameDT=off
  Alive50_inc : Sum  OutDataTypeStr=uint8
  Alive50_one : Constant  OutDataTypeStr=uint8  SampleTime=-1
  Alive50_prev : UnitDelay  SampleTime=-1
  Heartbeat : simulink/Sources/Counter Free-Running  NumBits=8  tsamp=Ts.comm
  Impl_type_u8 : DataTypeConversion  OutDataTypeStr=uint8  RndMeth=Round
  Implement_Aux : Subsystem  ReferencedSubsystem=fw_implement_aux
  Link_ok : Logic  Operator=NOT  Inputs=1  AllPortsSameDT=off  OutDataTypeStr=boolean
  Platform_BC : BusCreator  Inputs=8
  Sel_adc : BusSelector  OutputSignals=T_encl
  Sel_bms_chg : BusSelector  OutputSignals=bms.charging
  Sel_bms_hv : BusSelector  OutputSignals=bms.hv_ready
  Sel_fi_stall : BusSelector  OutputSignals=fault_inject
  Sel_fw_bms : BusSelector  OutputSignals=bms
  Sel_fw_st : BusSelector  OutputSignals=st,di_word
  Sel_impl_ready : BusSelector  OutputSignals=ready
  Sel_impl_type : BusSelector  OutputSignals=impl_type
  Sel_st_link : BusSelector  OutputSignals=st.rc.rc_link_lost
  Sel_st_lq : BusSelector  OutputSignals=st.rc.lq
  Sel_st_s02 : BusSelector  OutputSignals=st.mode,st.cmd_src,st.rc.rc_mode_sw,st.rc.rc_aux_cmd,st.rc.rc_aux_seq
  Sel_st_s08 : BusSelector  OutputSignals=st.rc.failsafe,st.estop_active,st.drive_ready
  Sel_st_s17 : BusSelector  OutputSignals=st.fault_word,st.warn_word,st.drive_fault_word,st.v_track_LR
  Sel_st_vc : BusSelector  OutputSignals=st.vc_tel
  Sel_st_wdg : BusSelector  OutputSignals=st.wdg_reset_seen
  Stall50 : simulink/Logic and Bit Operations/Compare To Zero  relop=~=  OutDataTypeStr=boolean
  Stall50_mask : simulink/Logic and Bit Operations/Bitwise Operator  logicop=AND  UseBitMask=on  BitMask=2  BitMaskRealWorld=Stored Integer
  Status_BC : BusCreator  Inputs=26  OutDataTypeStr=Bus: Bus_McuStatus  NonVirtualBus=on
      settings: InheritFromInputs=off
  T_mcu_na : Constant  Value=0  OutDataTypeStr=double  SampleTime=Ts.comm
  V_applied : Selector  InputPortWidth=11  IndexOptions=Index vector (dialog)  Indices=3  OutputSizes=1
  Valid : Constant  Value=true  OutDataTypeStr=boolean  SampleTime=Ts.comm
  W_applied : Selector  InputPortWidth=11  IndexOptions=Index vector (dialog)  Indices=4  OutputSizes=1
  do_aux : Outport
  pwm_duty : Outport  Port=2
  impl_enable : Outport  Port=3
  impl_fault_reset : Outport  Port=4
  impl_speed_rpm : Outport  Port=5
  status : Outport  Port=6
  alive50 : Outport  Port=7
  adc : Outport  Port=8
  wires:
  adc_raw/1 -> ADC_Scaling/1  "adc_raw"
  mcu_temp_degC/1 -> ADC_Scaling/2  "mcu_temp_degC"
  rt50/1 -> Sel_st_lq/1, Sel_fi_stall/1, Sel_st_s17/1, Sel_st_vc/1, Sel_st_wdg/1, Sel_bms_chg/1, Sel_bms_hv/1, Sel_st_s08/1, Sel_st_link/1, Sel_fw_st/1, Sel_st_s02/1, Sel_fw_bms/1  "rt50"
  gnc_cmd/1 -> Platform_BC/3  "gnc_cmd"
  comp_ok/1 -> Platform_BC/4  "comp_ok"
  comp_age/1 -> Platform_BC/5, Age_ms/1  "comp_age"
  impl/1 -> Platform_BC/7, Sel_impl_type/1, Sel_impl_ready/1  "impl"
  Sel_st_link/1 -> Link_ok/1  "<rc_link_lost>"
  Sel_fi_stall/1 -> Stall50_mask/1  "<fault_inject>"
  Sel_st_vc/1 -> W_applied/1, V_applied/1  "<vc_tel>"
  Link_ok/1 -> Status_BC/7  "rc_link_ok"
  Age_ms/1 -> Age_ms_u16/1  "Age_ms"
  Alive50_one/1 -> Alive50_inc/2  "Alive50_one"
  Stall50_mask/1 -> Stall50/1  "Stall50_mask"
  ADC_Scaling/1 -> adc/1, Sel_adc/1, Platform_BC/6  "adc"
  Sel_fw_st/1 -> Platform_BC/1  "<st>"
  Sel_fw_st/2 -> Platform_BC/2  "<di_word>"
  Sel_fw_bms/1 -> Platform_BC/8  "<bms>"
  Sel_impl_type/1 -> Impl_type_u8/1  "<impl_type>"
  Platform_BC/1 -> Implement_Aux/1  "fw50"
  Alive50_inc/1 -> Alive50/3  "Alive50_inc"
  T_mcu_na/1 -> Status_BC/1  "t_mcu"
  Heartbeat/1 -> Status_BC/16  "heartbeat"
  Valid/1 -> Status_BC/26  "valid"
  Stall50/1 -> Alive50/2  "Stall50"
  V_applied/1 -> Status_BC/21  "v_applied"
  W_applied/1 -> Status_BC/22  "w_applied"
  Impl_type_u8/1 -> Status_BC/15  "implement_type"
  Age_ms_u16/1 -> Status_BC/23  "gnc_cmd_age_ms"
  Sel_st_s02/1 -> Status_BC/2  "<mode>"
  Sel_st_s02/2 -> Status_BC/3  "<cmd_src>"
  Sel_st_s02/3 -> Status_BC/4  "<rc_mode_sw>"
  Sel_st_s02/4 -> Status_BC/5  "<rc_aux_cmd>"
  Sel_st_s02/5 -> Status_BC/6  "<rc_aux_seq>"
  Sel_st_s08/1 -> Status_BC/8  "<failsafe>"
  Sel_st_s08/2 -> Status_BC/9  "<estop_active>"
  Sel_st_s08/3 -> Status_BC/10  "<drive_ready>"
  Sel_bms_hv/1 -> Status_BC/11  "<hv_ready>"
  Sel_impl_ready/1 -> Status_BC/12  "<ready>"
  Sel_bms_chg/1 -> Status_BC/13  "<charging>"
  Sel_st_wdg/1 -> Status_BC/14  "<wdg_reset_seen>"
  Sel_st_s17/1 -> Status_BC/17  "<fault_word>"
  Sel_st_s17/2 -> Status_BC/18  "<warn_word>"
  Sel_st_s17/3 -> Status_BC/19  "<drive_fault_word>"
  Sel_st_s17/4 -> Status_BC/20  "<v_track_LR>"
  Sel_st_lq/1 -> Status_BC/24  "<lq>"
  Sel_adc/1 -> Status_BC/25  "<T_encl>"
  Status_BC/1 -> status/1  "status"
  Alive50/1 -> alive50/1, Alive50_prev/1  "alive50"
  Implement_Aux/1 -> do_aux/1  "do_aux"
  Implement_Aux/2 -> pwm_duty/1  "pwm_duty"
  Implement_Aux/3 -> impl_enable/1  "impl_enable"
  Implement_Aux/4 -> impl_fault_reset/1  "impl_fault_reset"
  Implement_Aux/5 -> impl_speed_rpm/1  "impl_speed_rpm"
  Alive50_prev/1 -> Alive50_inc/1, Alive50/1  "Alive50_prev"
